simulink model "admittance_1d"  (R2025b)
settings: Solver=ode45  StartTime=0.0  StopTime=1.5  RelTol=1e-3
undefined symbols (not defined in the file): dspblkCoreblockFVToolHelper, gcbh
settings Model: Creator=Compu  LastModifiedBy=Compu

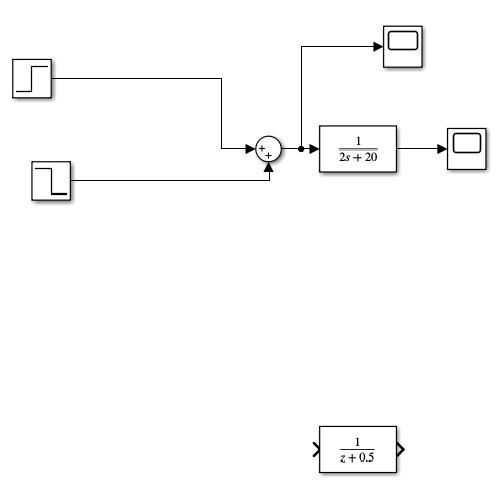
[thumbnail: Simulink's stored preview of the top-level diagram]
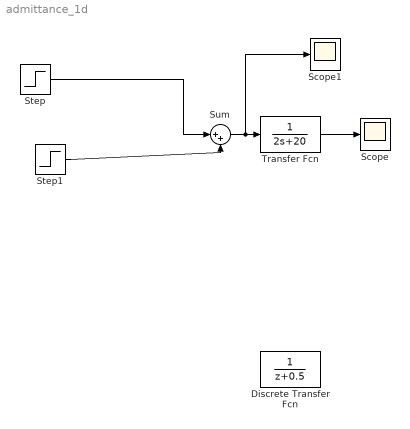
== system admittance_1d ==
  Discrete Transfer Fcn : DiscreteTransferFcn  LoadFcn=dspblkCoreblockFVToolHelper(gcbh,'load');
      settings: CopyFcn=dspblkCoreblockFVToolHelper(gcbh,'copy');  DeleteFcn=dspblkCoreblockFVToolHelper(gcbh,'close');  ModelCloseFcn=dspblkCoreblockFVToolHelper(gcbh,'close');  PreSaveFcn=dspblkCoreblockFVToolHelper(gcbh,'presave');  PostSaveFcn=dspblkCoreblockFVToolHelper(gcbh,'postsave');  CloseFcn=dspblkCoreblockFVToolHelper(gcbh,'close');
  Scope : Scope
      settings: ActiveDisplayYMinimum=-0.062078876313007215  ActiveDisplayYMaximum=0.558709886817065
  Scope1 : Scope
      settings: ActiveDisplayYMinimum=-1.2499999999999998  ActiveDisplayYMaximum=11.25
  Step : Step  Time=0  After=10  SampleTime=0
  Step1 : Step  Time=0.5  After=-10  SampleTime=0
  Sum : Sum  Inputs=|++
  Transfer Fcn : TransferFcn  Denominator=[2 20]
  wires:
  Sum/1 -> Scope1/1, Transfer Fcn/1
  Step/1 -> Sum/1
  Step1/1 -> Sum/2
  Transfer Fcn/1 -> Scope/1
